simulink model "s1_stima_ideale"  (R2025b)
settings: Solver=ode45  StartTime=0.0  StopTime=50  FixedStep=1  RelTol=1e-3
settings Model: Creator=sciau  LastModifiedBy=sciau

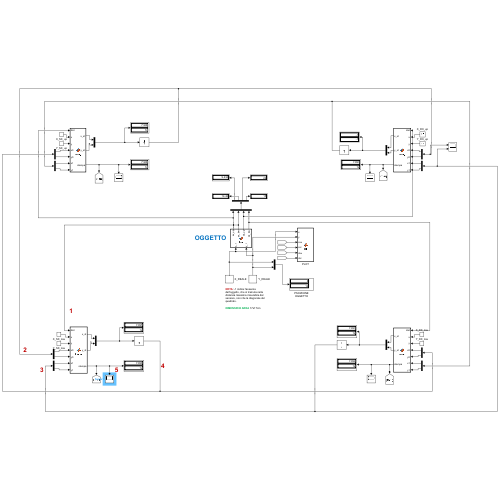
[thumbnail: Simulink's stored preview of the top-level diagram]
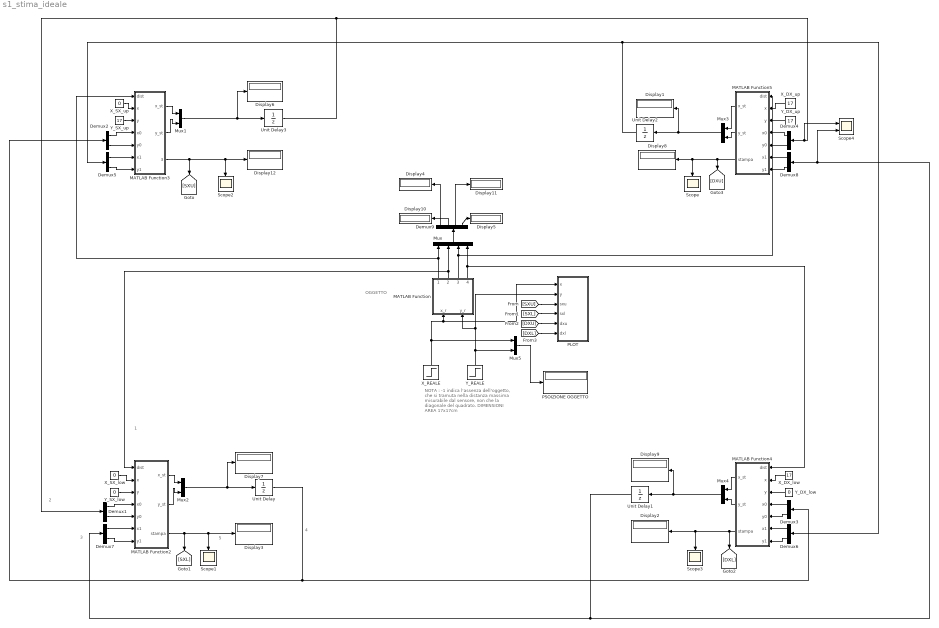
== system s1_stima_ideale ==
  note: 1
  note: OGGETTO
  note: NOTA : -1 indica l'assenza dell'oggetto, che si tramuta nella distanza massima misurabile dal sensore, non che la diagonale del quadrato.
      |
      | DIMENSIONI AREA 17x17cm
  note: 2
  note: 3
  note: 4
  note: 5
  Demux{1..8} (8 alike) : Demux  Outputs=2
  Demux9 : Demux
  Display{1..12} (12 alike) : Display
  MATLAB Function : MATLAB Function  TreatAsAtomicUnit=on
  MATLAB Function2 : MATLAB Function  TreatAsAtomicUnit=on
  MATLAB Function3 : MATLAB Function  TreatAsAtomicUnit=on
  MATLAB Function4 : MATLAB Function  TreatAsAtomicUnit=on
  MATLAB Function5 : MATLAB Function  TreatAsAtomicUnit=on
  Mux : Mux
  Mux{1..5} (5 alike) : Mux  Inputs=2
  PLOT : MATLAB Function  TreatAsAtomicUnit=on
  PSOIZIONE OGGETTO : Display
  Scope{,1..3} (4 alike) : Scope
      Scope settings: ActiveDisplayYMinimum=-1  ActiveDisplayYMaximum=1
      Scope1 settings: ActiveDisplayYMinimum=-3.2499999999999996  ActiveDisplayYMaximum=19.25
      Scope2 settings: ActiveDisplayYMinimum=-1  ActiveDisplayYMaximum=1  DataLoggingVariableName=ScopeData2
      Scope3 settings: ActiveDisplayYMinimum=-1  ActiveDisplayYMaximum=1  DataLoggingVariableName=ScopeData3
  Scope4 : Scope  NumInputPorts=2
      settings: ActiveDisplayYMinimum=-1  ActiveDisplayYMaximum=1  DataLoggingVariableName=ScopeData4
  Unit Delay{,1..3} (4 alike) : UnitDelay  SampleTime=-1  HasFrameUpgradeWarning=on
  X_DX_low : Constant  Value=17
  X_DX_up : Constant  Value=17
  X_REALE : Step  Before=-1  After=8  SampleTime=0
  X_SX_low : Constant  Value=0
  X_SX_up : Constant  Value=0
  Y_DX_low : Constant  Value=0
  Y_DX_up : Constant  Value=17
  Y_REALE : Step  Before=-1  After=12  SampleTime=0
  Y_SX_low : Constant  Value=0
  Y_SX_up : Constant  Value=17
  wires:
  X_REALE/1 -> MATLAB Function/1(x_r), PLOT/1(x), Mux5/1
  Y_REALE/1 -> MATLAB Function/2(y_r), PLOT/2(y), Mux5/2
  MATLAB Function/1(sx_up) -> MATLAB Function3/1(dist), Mux/1
  MATLAB Function/2(sx_low) -> MATLAB Function2/1(dist), Mux/2
  MATLAB Function/3(dx_up) -> MATLAB Function5/1(dist), Mux/3
  MATLAB Function/4(dx_low) -> Mux/4, MATLAB Function4/1(dist)
  X_SX_low/1 -> MATLAB Function2/2(x)
  Y_SX_low/1 -> MATLAB Function2/3(y)
  X_SX_up/1 -> MATLAB Function3/2(x)
  Y_SX_up/1 -> MATLAB Function3/3(y)
  MATLAB Function3/1(x_st) -> Mux1/1
  MATLAB Function3/2(y_st) -> Mux1/2
  Mux1/1 -> Display6/1, Unit Delay3/1
  Demux1/1 -> MATLAB Function2/4(x0)
  Demux1/2 -> MATLAB Function2/5(y0)
  X_DX_low/1 -> MATLAB Function4/2(x)
  Y_DX_low/1 -> MATLAB Function4/3(y)
  MATLAB Function2/1(x_st) -> Mux2/1
  MATLAB Function2/2(y_st) -> Mux2/2
  Mux2/1 -> Unit Delay/1, Display7/1
  Demux2/1 -> MATLAB Function3/4(x0)
  Demux2/2 -> MATLAB Function3/5(y0)
  Demux3/1 -> MATLAB Function4/4(x0)
  Y_DX_up/1 -> MATLAB Function5/3(y)
  Demux4/1 -> MATLAB Function5/4(x0)
  X_DX_up/1 -> MATLAB Function5/2(x)
  Demux4/2 -> MATLAB Function5/5(y0)
  MATLAB Function5/1(x_st) -> Mux3/1
  MATLAB Function5/2(y_st) -> Mux3/2
  Mux3/1 -> Display1/1, Unit Delay2/1
  Demux5/1 -> MATLAB Function3/6(x1)
  Demux5/2 -> MATLAB Function3/7(y1)
  Demux3/2 -> MATLAB Function4/5(y0)
  Demux6/1 -> MATLAB Function4/6(x1)
  Demux6/2 -> MATLAB Function4/7(y1)
  MATLAB Function4/1(x_st) -> Mux4/1
  Demux7/1 -> MATLAB Function2/6(x1)
  Demux7/2 -> MATLAB Function2/7(y1)
  Demux8/1 -> MATLAB Function5/6(x1)
  Demux8/2 -> MATLAB Function5/7(y1)
  Mux4/1 -> Display9/1, Unit Delay1/1
  Unit Delay/1 -> Demux2/1, Demux3/1
  Unit Delay1/1 -> Demux7/1, Scope4/2, Demux8/1
  Unit Delay2/1 -> Demux6/1, Demux5/1
  Unit Delay3/1 -> Scope4/1, Demux4/1, Demux1/1
  Mux5/1 -> PSOIZIONE OGGETTO/1
  [SXU] -> PLOT/3(sxu)
  [DXL] -> PLOT/6(dxl)
  [DXU] -> PLOT/5(dxu)
  [SXL] -> PLOT/4(sxl)
  Mux/1 -> Demux9/1
  Demux9/2 -> Display10/1
  Demux9/3 -> Display11/1
  Demux9/1 -> Display4/1
  Demux9/4 -> Display5/1
  MATLAB Function5/3(stampa) -> Scope/1, Display8/1, [DXU]
  MATLAB Function4/3(stampa) -> [DXL], Scope3/1, Display2/1
  MATLAB Function4/2(y_st) -> Mux4/2
  MATLAB Function3/3(stampa) -> [SXU], Scope2/1, Display12/1
  MATLAB Function2/3(stampa) -> Display3/1, Scope1/1, [SXL]

== matlab function s1_stima_ideale/PLOT ==
  data: x input; y input; sxu input; sxl input; dxu input; dxl input
function dis(x,y,sxu,sxl,dxu,dxl)

    % Mantieni il grafico attivo tra le chiamate
    persistent firstRun
    if isempty(firstRun)
        firstRun = true;
    end

    % --- Disegno iniziale del quadrato (solo la prima volta) ---
    if firstRun
        clf;
        axis equal;
        grid on;
        hold on;
        % Centro del quadrato
        cx = 8.5;
        cy = 8.5;
        L = 17;

        % Vertici del quadrato
        X = [cx-L/2, cx+L/2, cx+L/2, cx-L/2, cx-L/2];
        Y = [cy-L/2, cy-L/2, cy+L/2, cy+L/2, cy-L/2];

        plot(X, Y, 'b-', 'LineWidth', 2);
        firstRun = false;
    end

    % --- Disegno dei punti SOLO quando cambiano valore ---
    if x > -1 && y > -1
        plot(x, y, 'ro', 'MarkerSize', 10, 'LineWidth', 2);
        plot(sxu(1), sxu(2), 'go', 'MarkerSize', 3, 'LineWidth', 2);
        plot(sxl(1), sxl(2), 'mo', 'MarkerSize', 3, 'LineWidth', 2);
        plot(dxu(1), dxu(2), 'co', 'MarkerSize', 3, 'LineWidth', 2);
        plot(dxl(1), dxl(2), 'yo', 'MarkerSize', 3, 'LineWidth', 2);
    end


end

== matlab function s1_stima_ideale/MATLAB Function ==
  data: x_r input; sx_up output; y_r input; sx_low output; dx_up output; dx_low output
function [sx_up, sx_low, dx_up, dx_low]= fcn(x_r, y_r)

if x_r==-1 && y_r==-1
        sx_up=22;
        sx_low=22;
        dx_low=22;
        dx_up=22;
else    

    %sensore in (0,0)
    %0=a*0+q->q=0
    %y_r=a*x_r+0

    a=y_r/x_r;
    %vedo se è nel range di coefficienti angolari per 
    %cui il punto è nel cono di visione
    if a>tand(30) && a<tand(60)
        sx_low=sqrt((0-x_r)^2+(0-y_r)^2);
    else
        sx_low=22;
    end

    %sensore in (17,17)
    %17=a*17+q->q=17-a*17
    %y_r=a*x_r+q=a*x_r+17-a*17
    
    a=(y_r-17)/(x_r-17);
    %vedo se è nel range di coefficienti angolari per 
    %cui il punto è nel cono di visione
    if a>tand(30) && a<tand(60)
        dx_up=sqrt((17-x_r)^2+(17-y_r)^2);
    else
        dx_up=22;
    end

    %sensore in (0,17)
    %17=a*0+q->q=17
    %y_r=a*x_r+q=a*x_r+17
    
    a=(y_r-17)/(x_r);
    %vedo se è nel range di coefficienti angolari per
    %cui il punto è nel cono di visione
    if a>tand(120) && a<tand(150)
        sx_up=sqrt((0-x_r)^2+(17-y_r)^2);
    else
        sx_up=22;
    end

    %sensore in (17,0)
    %0=a*17+q->q=-a17
    %y_r=a*x_r+q=a*x_r-a17
    
    a=(y_r)/(x_r-17);
    %vedo se è nel range di coefficienti angolari per 
    %cui il punto è nel cono di visione
    if a>tand(120) && a<tand(150)
        dx_low=sqrt((17-x_r)^2+(0-y_r)^2);
    else
        dx_low=22;
    end
end

end

== matlab function s1_stima_ideale/MATLAB Function2 ==
  data: dist input; x input; y input; x_st output; y_st output; x0 input; y0 input; x1 input; y1 input; stampa output
function [x_st, y_st,stampa] = triang(dist,x,y, x0, y0,x1,y1)    
    persistent xst
    persistent yst;
    if isempty(xst) && isempty(yst)
        % xst=8.5;
        % yst=8.5;
        xst=0.1;
        yst=0.1;
    end
        
    if dist<=20  
        x_st=xst;
        y_st=yst;
        lo_vedo=1;
    else
        x_st=-1;
        y_st=-1;
        lo_vedo=0;
    end

    x_medio=xst;
    y_medio=yst;
    n=1;

    if x0~=-1
        x_medio=x_medio+x0;
        y_medio=y_medio+y0;
        n=n+1;
    end
    if x1~=-1
        x_medio=x_medio+x1;
        y_medio=y_medio+y1;
        n=n+1;
    end

    x_medio=x_medio/n;
    y_medio=y_medio/n;

    if lo_vedo==1
        rx = x_medio-x;
        ry = y_medio-y;
        r=sqrt(rx*rx+ry*ry);
        error=r-dist;
    
        ux=rx/r;
        uy=ry/r;
    
        xst = x_medio - 0.5 * error * ux;
        yst = y_medio - 0.5 * error * uy;
    else
        xst = x_medio;
        yst = y_medio;
    end

    stampa=[xst,yst];

end

== matlab function s1_stima_ideale/MATLAB Function3 ==
  data: dist input; x input; y input; x_st output; y_st output; x0 input; y0 input; x1 input; y1 input; stampa output
function [x_st, y_st,stampa] = triang(dist,x,y, x0, y0,x1,y1)

    
    persistent xst
    persistent yst;
    if isempty(xst) && isempty(yst)
        % xst=8.5;
        % yst=8.5;
        xst=0.1;
        yst=0.1;
    end
        
    if dist<=20  
        x_st=xst;
        y_st=yst;
        lo_vedo=1;
    else
        x_st=-1;
        y_st=-1;
        lo_vedo=0;
    end

    x_medio=xst;
    y_medio=yst;
    n=1;

    if x0~=-1
        x_medio=x_medio+x0;
        y_medio=y_medio+y0;
        n=n+1;
    end
    if x1~=-1
        x_medio=x_medio+x1;
        y_medio=y_medio+y1;
        n=n+1;
    end

    x_medio=x_medio/n;
    y_medio=y_medio/n;

    if lo_vedo==1
        rx = x_medio-x;
        ry = y_medio-y;
        r=sqrt(rx*rx+ry*ry);
        error=r-dist;
    
        ux=rx/r;
        uy=ry/r;
    
        xst = x_medio - 0.5 * error * ux;
        yst = y_medio - 0.5 * error * uy;
    else
        xst = x_medio;
        yst = y_medio;
    end

    stampa=[xst,yst];

end

== matlab function s1_stima_ideale/MATLAB Function4 ==
  data: dist input; x input; y input; x_st output; y_st output; x0 input; y0 input; x1 input; y1 input; stampa output
function [x_st, y_st,stampa] = triang(dist,x,y, x0, y0,x1,y1)

    
    persistent xst
    persistent yst;
    if isempty(xst) && isempty(yst)
        % xst=8.5;
        % yst=8.5;
        xst=0.1;
        yst=0.1;
    end
        
    if dist<=20  
        x_st=xst;
        y_st=yst;
        lo_vedo=1;
    else
        x_st=-1;
        y_st=-1;
        lo_vedo=0;
    end

    x_medio=xst;
    y_medio=yst;
    n=1;

    if x0~=-1
        x_medio=x_medio+x0;
        y_medio=y_medio+y0;
        n=n+1;
    end
    if x1~=-1
        x_medio=x_medio+x1;
        y_medio=y_medio+y1;
        n=n+1;
    end

    x_medio=x_medio/n;
    y_medio=y_medio/n;

    if lo_vedo==1
        rx = x_medio-x;
        ry = y_medio-y;
        r=sqrt(rx*rx+ry*ry);
        error=r-dist;
    
        ux=rx/r;
        uy=ry/r;
    
        xst = x_medio - 0.5 * error * ux;
        yst = y_medio - 0.5 * error * uy;
    else
        xst = x_medio;
        yst = y_medio;
    end

    stampa=[xst,yst];

end

== matlab function s1_stima_ideale/MATLAB Function5 ==
  data: dist input; x input; y input; x_st output; y_st output; x0 input; y0 input; x1 input; y1 input; stampa output
function [x_st, y_st,stampa] = triang(dist,x,y, x0, y0,x1,y1)

    
    persistent xst
    persistent yst;
    if isempty(xst) && isempty(yst)
        % xst=8.5;
        % yst=8.5;
        xst=0.1;
        yst=0.1;
    end
        
    if dist<=20  
        x_st=xst;
        y_st=yst;
        lo_vedo=1;
    else
        x_st=-1;
        y_st=-1;
        lo_vedo=0;
    end

    x_medio=xst;
    y_medio=yst;
    n=1;

    if x0~=-1
        x_medio=x_medio+x0;
        y_medio=y_medio+y0;
        n=n+1;
    end
    if x1~=-1
        x_medio=x_medio+x1;
        y_medio=y_medio+y1;
        n=n+1;
    end

    x_medio=x_medio/n;
    y_medio=y_medio/n;

    if lo_vedo==1
        rx = x_medio-x;
        ry = y_medio-y;
        r=sqrt(rx*rx+ry*ry);
        error=r-dist;
    
        ux=rx/r;
        uy=ry/r;
    
        xst = x_medio - 0.5 * error * ux;
        yst = y_medio - 0.5 * error * uy;
    else
        xst = x_medio;
        yst = y_medio;
    end

    stampa=[xst,yst];

end
